simulink model "hdlcoderviterbi2"  (R2026a)
settings: Solver=VariableStepDiscrete  StopTime=8000
PreLoadFcn:
  | EsNo = 0;
libraries: commsink2 x3, commdigbbndpm3 x2, commcnvcod2 x2, commchan3 x1, commrandsrc3 x1, simulink x1
(part 1 of 2)
Description:
  | Viterbi Decoder Using the MATLAB(R) Function Block
  | This example shows how to use HDL Coder(TM) to check, generate,
  | and verify HDL for a fixed-point Viterbi decoder model built using the
  | MATLAB Function Block.
settings Model: ExtModeAutoUpdateStatusClock=off  Creator=The MathWorks, Inc.  LastModifiedBy=The MathWorks, Inc.
settings OptimizationCC: ConditionallyExecuteInputs=off  InitFltsAndDblsToZero=on  EfficientMapNaN2IntZero=off
settings DebuggingCC: AlgebraicLoopMsg=error  SignalResolutionControl=TryResolveAllWithWarning  MultiTaskDSMMsg=warning  SingleTaskRateTransMsg=error  IntegerOverflowMsg=none  ParameterPrecisionLossMsg=none  SymbolicDimsDataTypeCodeGenerationDiagnostic=none  IntegerSaturationMsg=none
settings HardwareCC: ProdHWDeviceType=ASIC/FPGA  ProdEqTarget=off
settings GRTTargetCC: CombineOutputUpdateFcns=off  GRTInterface=on

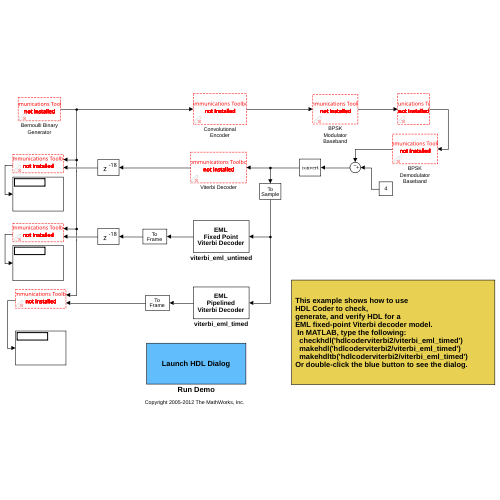
[thumbnail: Simulink's stored preview of the top-level diagram]
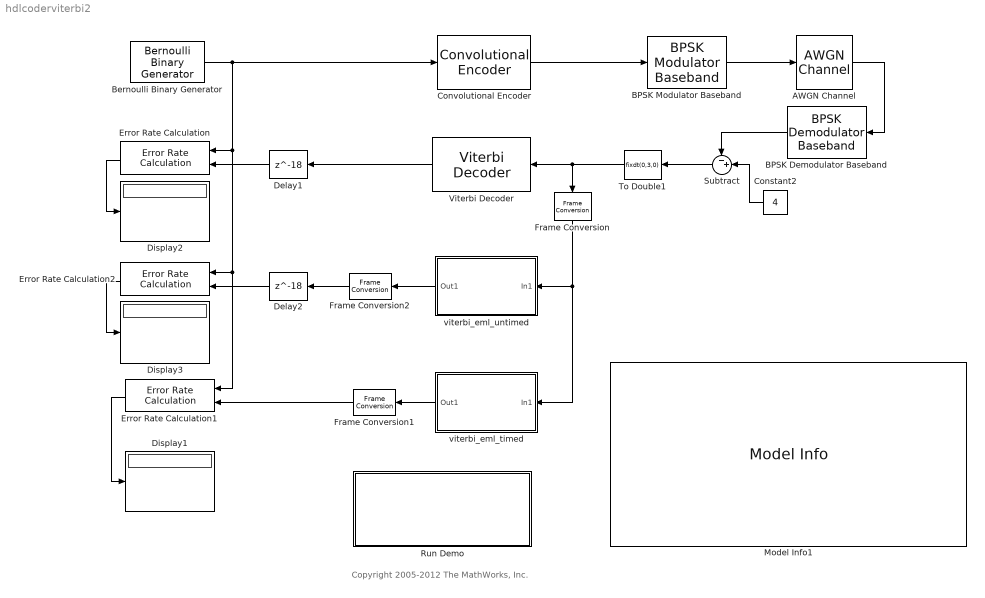
== system hdlcoderviterbi2 ==
  note: Copyright 2005-2012 The MathWorks, Inc.
  AWGN Channel : commchan3/AWGN Channel  LegacyMode=off  NoiseMethod="Signal to noise ratio  (Es/No)"  noiseMode="Signal to noise ratio  (SNR)"  EbNo=10  EsNo=EsNo  SNR=10  BitsPerSymbol=1  SignalPower=1  SamplesPerSymbol=round(0.5 / 5.000000e-01)  SymbolPeriod=0.5  VarianceSource=Parameter  Variance=1  RandomStream=mt19937ar with seed  Seed=123456  SimulateUsing=Code generation
  BPSK Demodulator Baseband : commdigbbndpm3/BPSK Demodulator Baseband  DecType=Log-likelihood ratio  VarSource=Dialog  Variance=10^(-0.1*EsNo)  Ph=0  outDtype=double  derotateFactorWordLen=16  derotateFactorDataTypeStr=Inherit: Same word length as input  derotateFactorLastDataTypeStr=Inherit: Same word length as input
  BPSK Modulator Baseband : commdigbbndpm3/BPSK Modulator Baseband  Ph=0  outDtype=double  outWordLen=16  outUDDataType=sfix(16)  outFracLenMode=Best precision  outFracLen=15  outDataTypeStr=double  outLastDataTypeStr=double
  Bernoulli Binary Generator : commrandsrc3/Bernoulli Binary Generator  ProbabilityOfZero=0.5  SeedSource=Parameter  Seed=610  SampleTime=1  SamplesPerFrame=1  OutputDataType=boolean  SimulateUsing=Interpreted execution
  Constant2 : Constant  Value=4  OutDataTypeStr=Inherit: Inherit via back propagation
  Convolutional Encoder : commcnvcod2/Convolutional Encoder  trellis=poly2trellis(7, [171 133])  opMode=Continuous  DelayedResetAction=off  hasIniStPort=off  hasFinStPort=off  usePuncVector=off  punctureVector=[1; 1; 0; 1; 0; 1]  reset=Unused parameter value
  Delay1 : Delay  DelayLength=18  InitialCondition=0  InputProcessing=Columns as channels (frame based)
  Delay2 : Delay  DelayLength=18  InitialCondition=0  InputProcessing=Columns as channels (frame based)
  Display1 : Display
  Display2 : Display
  Display3 : Display
  Error Rate Calculation : commsink2/Error Rate Calculation  N=50  st_delay=100  cp_mode=Entire frame  subframe=[]  PMode=Port  WsName=BER_Data  RsMode2=off  stop=off  numErr=500  maxBits=1e6
  Error Rate Calculation1 : commsink2/Error Rate Calculation  N=50  st_delay=100  cp_mode=Entire frame  subframe=[]  PMode=Port  WsName=BER_Data  RsMode2=off  stop=off  numErr=100  maxBits=1e7
  Error Rate Calculation2 : commsink2/Error Rate Calculation  N=50  st_delay=100  cp_mode=Entire frame  subframe=[]  PMode=Port  WsName=BER_Data  RsMode2=off  stop=off  numErr=100  maxBits=1e7
  Frame Conversion : FrameConversion  OutFrame=Sample-based
  Frame Conversion1 : FrameConversion
  Frame Conversion2 : FrameConversion
  Model Info1 : simulink/Model-Wide Utilities/Model Info  Frame=on  DisplayStringWithTags=|  HorizontalTextAlignment=Left  LeftAlignmentValue=0.02
      | This example shows how to use
      | HDL Coder to check, 
      | generate, and verify HDL for a
      | EML fixed-point Viterbi decoder model.
      |  In MATLAB, type the following:
      |   checkhdl('hdlcoderviterbi2/viterbi_eml_timed')
      |   makehdl('hdlcoderviterbi2/viterbi_eml_timed')
      |   makehdltb('hdlcoderviterbi2/viterbi_eml_timed')
      | Or double-click the blue button to see the dialog.
  Run Demo : Subsystem
      settings: OpenFcn=hdldialog(bdroot)
      mask Display: disp('Launch HDL Dialog')
  Subtract : Sum  Inputs=-+|
  To Double1 : DataTypeConversion  OutDataTypeStr=fixdt(0,3,0)
  Viterbi Decoder : commcnvcod2/Viterbi Decoder  trellis=poly2trellis(7, [171 133])  isPunctured=off  punctureVector=[1; 1; 0; 1; 0; 1]  erasures=off  dectype=Soft decision  nsdecb=3  runSigValErrCheck=off  tbdepth=32  opmode=Continuous  reset=off  delayedResetAction=off  smWordLength=16  outDataType=boolean
  viterbi_eml_timed : Subsystem
      settings: RTWMemSecFuncInitTerm=Default  RTWMemSecFuncExecute=Default  RTWMemSecDataConstants=Default  RTWMemSecDataInternal=Default  RTWMemSecDataParameters=Default
      mask Display: disp('EML\nPipelined\nViterbi Decoder');
  viterbi_eml_untimed : Subsystem
      settings: RTWMemSecFuncInitTerm=Default  RTWMemSecFuncExecute=Default  RTWMemSecDataConstants=Default  RTWMemSecDataInternal=Default  RTWMemSecDataParameters=Default
      mask Display: disp('EML\nFixed Point\nViterbi Decoder');
  wires:
  Bernoulli Binary Generator/1 -> Error Rate Calculation/1, Error Rate Calculation2/1, Error Rate Calculation1/1, Convolutional Encoder/1
  BPSK Modulator Baseband/1 -> AWGN Channel/1
  Convolutional Encoder/1 -> BPSK Modulator Baseband/1
  viterbi_eml_untimed/1(Out1) -> Frame Conversion2/1
  Viterbi Decoder/1 -> Delay1/1
  Subtract/1 -> To Double1/1
  To Double1/1 -> Viterbi Decoder/1, Frame Conversion/1
  Frame Conversion/1 -> viterbi_eml_untimed/1(In1), viterbi_eml_timed/1(In1)
  Frame Conversion2/1 -> Delay2/1
  viterbi_eml_timed/1(Out1) -> Frame Conversion1/1
  Frame Conversion1/1 -> Error Rate Calculation1/2
  Delay1/1 -> Error Rate Calculation/2
  Delay2/1 -> Error Rate Calculation2/2
  Error Rate Calculation/1 -> Display2/1
  Error Rate Calculation2/1 -> Display3/1
  Error Rate Calculation1/1 -> Display1/1
  AWGN Channel/1 -> BPSK Demodulator Baseband/1
  BPSK Demodulator Baseband/1 -> Subtract/1
  Constant2/1 -> Subtract/2

== system hdlcoderviterbi2/Run Demo ==

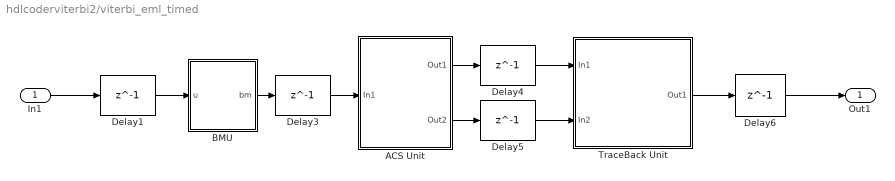
== system hdlcoderviterbi2/viterbi_eml_timed ==
  In1 : Inport
  ACS Unit : Subsystem
      settings: RTWMemSecFuncInitTerm=Default  RTWMemSecFuncExecute=Default  RTWMemSecDataConstants=Default  RTWMemSecDataInternal=Default  RTWMemSecDataParameters=Default
  BMU : MATLAB Function  TreatAsAtomicUnit=on
  Delay{1,3..6} (5 alike) : Delay  DelayLength=1  InitialCondition=0  UseCircularBuffer=on
  TraceBack Unit : Subsystem
  Out1 : Outport  VectorParamsAs1DForOutWhenUnconnected=off
  wires:
  In1/1 -> Delay1/1
  ACS Unit/1(Out1) -> Delay4/1
  ACS Unit/2(Out2) -> Delay5/1
  TraceBack Unit/1(Out1) -> Delay6/1
  BMU/1(bm) -> Delay3/1
  Delay1/1 -> BMU/1(u)
  Delay3/1 -> ACS Unit/1(In1)
  Delay4/1 -> TraceBack Unit/1(In1)
  Delay5/1 -> TraceBack Unit/2(In2)
  Delay6/1 -> Out1/1

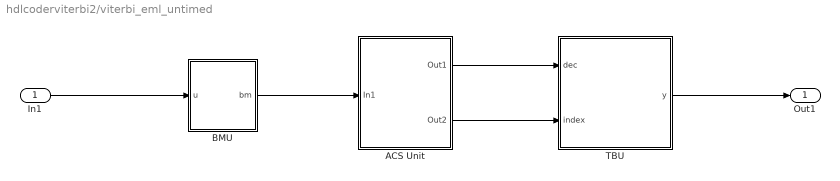
== system hdlcoderviterbi2/viterbi_eml_untimed ==
  In1 : Inport
  ACS Unit : Subsystem
      settings: RTWMemSecFuncInitTerm=Default  RTWMemSecFuncExecute=Default  RTWMemSecDataConstants=Default  RTWMemSecDataInternal=Default  RTWMemSecDataParameters=Default
  BMU : MATLAB Function  TreatAsAtomicUnit=on
  TBU : MATLAB Function  TreatAsAtomicUnit=on
  Out1 : Outport  VectorParamsAs1DForOutWhenUnconnected=off
  wires:
  In1/1 -> BMU/1(u)
  ACS Unit/1(Out1) -> TBU/1(dec)
  ACS Unit/2(Out2) -> TBU/2(index)
  TBU/1(y) -> Out1/1
  BMU/1(bm) -> ACS Unit/1(In1)

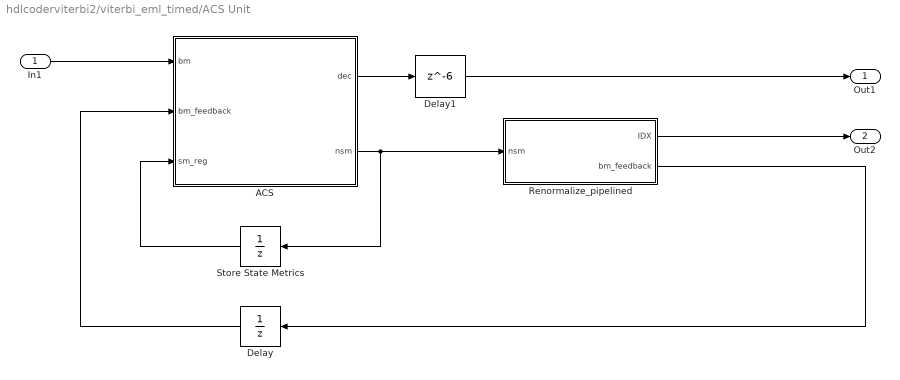
== system hdlcoderviterbi2/viterbi_eml_timed/ACS Unit ==
  In1 : Inport
  ACS : MATLAB Function  TreatAsAtomicUnit=on
  Delay : UnitDelay  SampleTime=-1
  Delay1 : Delay  DelayLength=6  InitialCondition=0
  Renormalize_pipelined : MATLAB Function  TreatAsAtomicUnit=on
  Store State Metrics : UnitDelay  SampleTime=-1
  Out1 : Outport  VectorParamsAs1DForOutWhenUnconnected=off
  Out2 : Outport  Port=2  VectorParamsAs1DForOutWhenUnconnected=off
  wires:
  Store State Metrics/1 -> ACS/3(sm_reg)
  ACS/1(dec) -> Delay1/1
  Delay/1 -> ACS/2(bm_feedback)
  In1/1 -> ACS/1(bm)
  ACS/2(nsm) -> Store State Metrics/1, Renormalize_pipelined/1(nsm)
  Renormalize_pipelined/2(bm_feedback) -> Delay/1
  Delay1/1 -> Out1/1
  Renormalize_pipelined/1(IDX) -> Out2/1

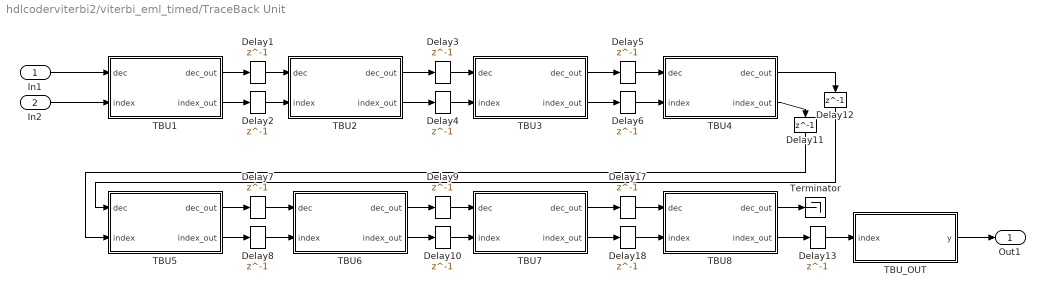
== system hdlcoderviterbi2/viterbi_eml_timed/TraceBack Unit ==
  In1 : Inport
  In2 : Inport  Port=2
  Delay{1..13,17..18} (15 alike) : Delay  DelayLength=1  InitialCondition=0  UseCircularBuffer=on
  TBU1 : MATLAB Function  TreatAsAtomicUnit=on
  TBU2 : MATLAB Function  TreatAsAtomicUnit=on
  TBU3 : MATLAB Function  TreatAsAtomicUnit=on
  TBU4 : MATLAB Function  TreatAsAtomicUnit=on
  TBU5 : MATLAB Function  TreatAsAtomicUnit=on
  TBU6 : MATLAB Function  TreatAsAtomicUnit=on
  TBU7 : MATLAB Function  TreatAsAtomicUnit=on
  TBU8 : MATLAB Function  TreatAsAtomicUnit=on
  TBU_OUT : MATLAB Function  TreatAsAtomicUnit=on
  Terminator : Terminator
  Out1 : Outport  VectorParamsAs1DForOutWhenUnconnected=off
  wires:
  In1/1 -> TBU1/1(dec)
  In2/1 -> TBU1/2(index)
  TBU4/2(index_out) -> Delay11/1
  TBU4/1(dec_out) -> Delay12/1
  TBU1/1(dec_out) -> Delay1/1
  TBU1/2(index_out) -> Delay2/1
  Delay1/1 -> TBU2/1(dec)
  Delay2/1 -> TBU2/2(index)
  Delay3/1 -> TBU3/1(dec)
  Delay4/1 -> TBU3/2(index)
  TBU2/1(dec_out) -> Delay3/1
  TBU2/2(index_out) -> Delay4/1
  TBU3/1(dec_out) -> Delay5/1
  TBU3/2(index_out) -> Delay6/1
  Delay5/1 -> TBU4/1(dec)
  Delay6/1 -> TBU4/2(index)
  TBU5/1(dec_out) -> Delay7/1
  TBU5/2(index_out) -> Delay8/1
  Delay7/1 -> TBU6/1(dec)
  Delay8/1 -> TBU6/2(index)
  Delay9/1 -> TBU7/1(dec)
  Delay10/1 -> TBU7/2(index)
  TBU6/1(dec_out) -> Delay9/1
  TBU6/2(index_out) -> Delay10/1
  TBU7/1(dec_out) -> Delay17/1
  TBU7/2(index_out) -> Delay18/1
  Delay17/1 -> TBU8/1(dec)
  Delay18/1 -> TBU8/2(index)
  Delay12/1 -> TBU5/1(dec)
  Delay11/1 -> TBU5/2(index)
  TBU8/1(dec_out) -> Terminator/1
  TBU8/2(index_out) -> Delay13/1
  Delay13/1 -> TBU_OUT/1(index)
  TBU_OUT/1(y) -> Out1/1

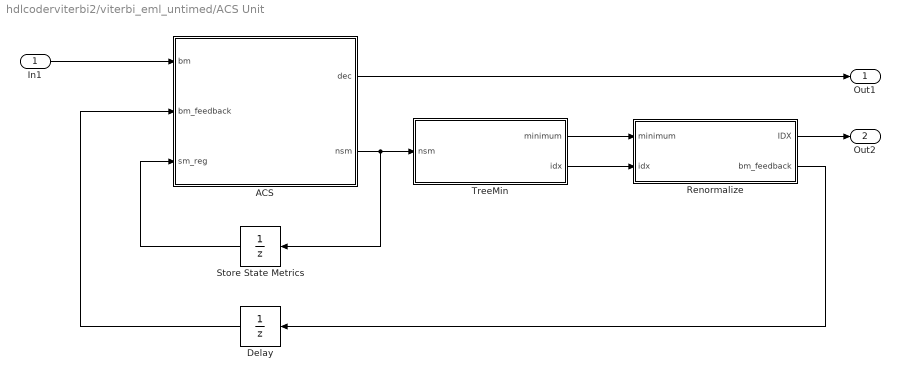
== system hdlcoderviterbi2/viterbi_eml_untimed/ACS Unit ==
  In1 : Inport
  ACS : MATLAB Function  TreatAsAtomicUnit=on
  Delay : UnitDelay  SampleTime=-1
  Renormalize : MATLAB Function  TreatAsAtomicUnit=on
  Store State Metrics : UnitDelay  SampleTime=-1
  TreeMin : MATLAB Function  TreatAsAtomicUnit=on
  Out1 : Outport  VectorParamsAs1DForOutWhenUnconnected=off
  Out2 : Outport  Port=2  VectorParamsAs1DForOutWhenUnconnected=off
  wires:
  Store State Metrics/1 -> ACS/3(sm_reg)
  ACS/1(dec) -> Out1/1
  Delay/1 -> ACS/2(bm_feedback)
  In1/1 -> ACS/1(bm)
  TreeMin/1(minimum) -> Renormalize/1(minimum)
  Renormalize/1(IDX) -> Out2/1
  ACS/2(nsm) -> TreeMin/1(nsm), Store State Metrics/1
  Renormalize/2(bm_feedback) -> Delay/1
  TreeMin/2(idx) -> Renormalize/2(idx)

== matlab function hdlcoderviterbi2/viterbi_eml_untimed/TBU ==
  settings: fimath=|
      | fimath(...
      | 'RoundMode', 'floor',...
      | 'OverflowMode', 'wrap',...
      | 'ProductMode', 'FullPrecision', 'ProductWordLength', 32,...
      | 'SumMode', 'FullPrecision', 'SumWordLength', 32,...
      | 'CastBeforeSum', true)
  data: dec input fixdt(0,1,0) size=[1 64]; index input fixdt(0,8,0) size=1; y output
function y = TBU(dec, index)

% traceback storage register
persistent tb_reg;  
if isempty(tb_reg)
    tb_reg = getfi(zeros(1,64), 0, 32, 0);
end

   
%--------------------------------------------------------------------------
% TBU (Trace Back Unit)
% Trace back unit restore the optimal path information stored in the 
% path metric register. The trace back depth of this decoder is 32 steps,
% which means every decoded symbol is based on the minimum path metric in the
% following 32 steps. 
%
% The trace back unit is implemented by a 32 stage shift register.
% Normal implementation uses 32 64-bit registers for trance back unit. 
% We use 64 32-bit registers instead because of the fixed-point bitwidth limit.
%--------------------------------------------------------------------------

% stores path metric decision inforamtion from PMU unit
tb_reg = bitconcat(bitsliceget(tb_reg, 31, 1), dec);

% trace back unit
for i=1:32
  index = tbunit(index, tb_reg, i);
end

% the 6th bit of the 32th trace back step is the decoder output
tband = bitget(index, 6);
y =  logical(tband);

end

%--------------------------------------------------------------------------
% TB Unit (Trace Back Unit)
% Given the index of the minimum metric node in the current stages,
% also given the stored decision information in the current stages,
% we can restore the index of the minimum metric node in the previous stage.
%--------------------------------------------------------------------------
function new_idx = tbunit (current_idx, tb_reg, stage)

idx = int32(current_idx) + int32(1);
tbread = bitget(tb_reg(idx), stage);

shift_idx = bitconcat(bitsliceget(current_idx, 5, 1), tbread);
new_idx = bitconcat(getfi(0, 0, 2, 0), shift_idx);

end


function myfi = getfi(input, issigned, wlen, flen)

fm = fimath(...
    'RoundMode', 'floor',...
    'OverflowMode', 'wrap',...
    'ProductMode', 'FullPrecision', 'ProductWordLength', 32,...
    'SumMode', 'FullPrecision', 'SumWordLength', 32,...
    'CastBeforeSum', true);

myfi = fi(input, issigned, wlen, flen, 'fimath', fm);

end

== matlab function hdlcoderviterbi2/viterbi_eml_timed/BMU ==
  settings: fimath=|
      | fimath(...
      | 'RoundMode', 'floor',...
      | 'OverflowMode', 'wrap',...
      | 'ProductMode', 'FullPrecision', 'ProductWordLength', 32,...
      | 'SumMode', 'FullPrecision', 'SumWordLength', 32,...
      | 'CastBeforeSum', true)
  data: u input fixdt(0,3,0) size=2; bm output
function bm = BMU(u)
%--------------------------------------------------------------------------
% Viterbi Decoder Demo
% 
% This model implements viterbi decoder in MATLAB Coder.
% The Viterbi Decoder block decodes fixed-point input symbols to produce 
% binary output symbols.
%--------------------------------------------------------------------------

% input symbol
u1 = u(1);
u2 = u(2);

%--------------------------------------------------------------------------
% BMC (Branch Metric) Unit
% This block calculates the Branch Metric (Hamming distance) of input symbols.
% The input are the quantized fixed-point symbols in the form of ufix3.

% Input Value   Interpretation
% 
% 0          Most confident zero
% 1          Second most confident zero
% 2          Third most confident zero
% 3          Least confident zero
% 4          Least confident one
% 5          Third most confident one
% 6          Second most confident one
% 7          Most confident one

%--------------------------------------------------------------------------

bm_max = getfi(7, 0, 3, 0);

bm_t1 = getfi(bm_max - u1, 0, 3, 0);
bm_t2 = getfi(bm_max - u2, 0, 3, 0);

bm = getfi(zeros(1,4), 0, 4, 0);

%----------------------------
bm(1) = u1 + u2; 

%----------------------------
bm(2) = u1 + bm_t2; 

%----------------------------
bm(3) = bm_t1 + u2;

%----------------------------
bm(4) = bm_t1 + bm_t2;

end

function myfi = getfi(input, issigned, wlen, flen)

fm = fimath(...
    'RoundMode', 'floor',...
    'OverflowMode', 'wrap',...
    'ProductMode', 'FullPrecision', 'ProductWordLength', 32,...
    'SumMode', 'FullPrecision', 'SumWordLength', 32,...
    'CastBeforeSum', true);

myfi = fi(input, issigned, wlen, flen, 'fimath', fm);

end

== matlab function hdlcoderviterbi2/viterbi_eml_timed/TraceBack Unit/TBU1 ==
  settings: fimath=|
      | fimath(...
      | 'RoundMode', 'floor',...
      | 'OverflowMode', 'wrap',...
      | 'ProductMode', 'FullPrecision', 'ProductWordLength', 32,...
      | 'SumMode', 'FullPrecision', 'SumWordLength', 32,...
      | 'CastBeforeSum', true)
  data: dec input fixdt(0,1,0) size=[1 64]; index input fixdt(0,8,0) size=1; dec_out output; index_out output
function [dec_out, index_out] = TBU(dec, index)
%--------------------------------------------------------------------------
% TBU (Trace Back Unit)
% Trace back unit restore the optimal path information stored in the 
% path metric register. The trace back depth of this decoder is 32 steps,
% which means every decoded symbol is based on the minimum path metric in the
% following 32 steps. 
%
% The trace back unit is implemented by a 32 stage shift register.
% In this pipelined model, 32 stage shift register is breaked into 8 4-stage shift registers. 
%--------------------------------------------------------------------------

% initialize 4-stage trace back storage shift register
persistent tb_reg1 tb_reg2 tb_reg3 tb_reg4
if isempty(tb_reg1)
    tb_reg1 = getfi(zeros(1, 64), 0, 1, 0);
end
if isempty(tb_reg2)
    tb_reg2 = getfi(zeros(1, 64), 0, 1, 0);
end
if isempty(tb_reg3)
    tb_reg3 = getfi(zeros(1, 64), 0, 1, 0);
end
if isempty(tb_reg4)
    tb_reg4 = getfi(zeros(1, 64), 0, 1, 0);
end

% 4-stage trace back storage shift register
% stores path metric decision inforamtion from ACS unit
dec_out = tb_reg4;
tb_reg4 = tb_reg3;
tb_reg3 = tb_reg2;
tb_reg2 = tb_reg1;
tb_reg1 = dec;

% stage one
idx = int32(index) + int32(1);
tbread = tb_reg1(idx);
shift_idx = bitconcat(bitsliceget(index, 5, 1), tbread);
index = bitconcat(getfi(0, 0, 2, 0), shift_idx);

% stage two
idx = int32(index) + int32(1);
tbread = tb_reg2(idx);
shift_idx = bitconcat(bitsliceget(index, 5, 1), tbread);
index = bitconcat(getfi(0, 0, 2, 0), shift_idx);

% stage three
idx = int32(index) + int32(1);
tbread = tb_reg3(idx);
shift_idx = bitconcat(bitsliceget(index, 5, 1), tbread);
index = bitconcat(getfi(0, 0, 2, 0), shift_idx);

% stage four
idx = int32(index) + int32(1);
tbread = tb_reg4(idx);
shift_idx = bitconcat(bitsliceget(index, 5, 1), tbread);
index_out = bitconcat(getfi(0, 0, 2, 0), shift_idx);

end

function myfi = getfi(input, issigned, wlen, flen)

fm = fimath(...
    'RoundMode', 'floor',...
    'OverflowMode', 'wrap',...
    'ProductMode', 'FullPrecision', 'ProductWordLength', 32,...
    'SumMode', 'FullPrecision', 'SumWordLength', 32,...
    'CastBeforeSum', true);

myfi = fi(input, issigned, wlen, flen, 'fimath', fm);

end

== matlab function hdlcoderviterbi2/viterbi_eml_timed/TraceBack Unit/TBU6 ==
  settings: fimath=|
      | fimath(...
      | 'RoundMode', 'floor',...
      | 'OverflowMode', 'wrap',...
      | 'ProductMode', 'FullPrecision', 'ProductWordLength', 32,...
      | 'SumMode', 'FullPrecision', 'SumWordLength', 32,...
      | 'CastBeforeSum', true)
  data: dec input fixdt(0,1,0) size=[1 64]; index input fixdt(0,8,0) size=1; dec_out output; index_out output
function [dec_out, index_out] = TBU(dec, index)
%--------------------------------------------------------------------------
% TBU (Trace Back Unit)
% Trace back unit restore the optimal path information stored in the 
% path metric register. The trace back depth of this decoder is 32 steps,
% which means every decoded symbol is based on the minimum path metric in the
% following 32 steps. 
%
% The trace back unit is implemented by a 32 stage shift register.
% In this pipelined model, 32 stage shift register is breaked into 8 4-stage shift registers. 
%--------------------------------------------------------------------------

% initialize 4-stage trace back storage shift register
persistent tb_reg1 tb_reg2 tb_reg3 tb_reg4
if isempty(tb_reg1)
    tb_reg1 = getfi(zeros(1, 64), 0, 1, 0);
end
if isempty(tb_reg2)
    tb_reg2 = getfi(zeros(1, 64), 0, 1, 0);
end
if isempty(tb_reg3)
    tb_reg3 = getfi(zeros(1, 64), 0, 1, 0);
end
if isempty(tb_reg4)
    tb_reg4 = getfi(zeros(1, 64), 0, 1, 0);
end

% 4-stage trace back storage shift register
% stores path metric decision inforamtion from ACS unit
dec_out = tb_reg4;
tb_reg4 = tb_reg3;
tb_reg3 = tb_reg2;
tb_reg2 = tb_reg1;
tb_reg1 = dec;

% stage one
idx = int32(index) + int32(1);
tbread = tb_reg1(idx);
shift_idx = bitconcat(bitsliceget(index, 5, 1), tbread);
index = bitconcat(getfi(0, 0, 2, 0), shift_idx);

% stage two
idx = int32(index) + int32(1);
tbread = tb_reg2(idx);
shift_idx = bitconcat(bitsliceget(index, 5, 1), tbread);
index = bitconcat(getfi(0, 0, 2, 0), shift_idx);

% stage three
idx = int32(index) + int32(1);
tbread = tb_reg3(idx);
shift_idx = bitconcat(bitsliceget(index, 5, 1), tbread);
index = bitconcat(getfi(0, 0, 2, 0), shift_idx);

% stage four
idx = int32(index) + int32(1);
tbread = tb_reg4(idx);
shift_idx = bitconcat(bitsliceget(index, 5, 1), tbread);
index_out = bitconcat(getfi(0, 0, 2, 0), shift_idx);

end

function myfi = getfi(input, issigned, wlen, flen)

fm = fimath(...
    'RoundMode', 'floor',...
    'OverflowMode', 'wrap',...
    'ProductMode', 'FullPrecision', 'ProductWordLength', 32,...
    'SumMode', 'FullPrecision', 'SumWordLength', 32,...
    'CastBeforeSum', true);

myfi = fi(input, issigned, wlen, flen, 'fimath', fm);

end

== matlab function hdlcoderviterbi2/viterbi_eml_timed/TraceBack Unit/TBU7 ==
  settings: fimath=|
      | fimath(...
      | 'RoundMode', 'floor',...
      | 'OverflowMode', 'wrap',...
      | 'ProductMode', 'FullPrecision', 'ProductWordLength', 32,...
      | 'SumMode', 'FullPrecision', 'SumWordLength', 32,...
      | 'CastBeforeSum', true)
  data: dec input fixdt(0,1,0) size=[1 64]; index input fixdt(0,8,0) size=1; dec_out output; index_out output
function [dec_out, index_out] = TBU(dec, index)
%--------------------------------------------------------------------------
% TBU (Trace Back Unit)
% Trace back unit restore the optimal path information stored in the 
% path metric register. The trace back depth of this decoder is 32 steps,
% which means every decoded symbol is based on the minimum path metric in the
% following 32 steps. 
%
% The trace back unit is implemented by a 32 stage shift register.
% In this pipelined model, 32 stage shift register is breaked into 8 4-stage shift registers. 
%--------------------------------------------------------------------------

% initialize 4-stage trace back storage shift register
persistent tb_reg1 tb_reg2 tb_reg3 tb_reg4
if isempty(tb_reg1)
    tb_reg1 = getfi(zeros(1, 64), 0, 1, 0);
end
if isempty(tb_reg2)
    tb_reg2 = getfi(zeros(1, 64), 0, 1, 0);
end
if isempty(tb_reg3)
    tb_reg3 = getfi(zeros(1, 64), 0, 1, 0);
end
if isempty(tb_reg4)
    tb_reg4 = getfi(zeros(1, 64), 0, 1, 0);
end

% 4-stage trace back storage shift register
% stores path metric decision inforamtion from ACS unit
dec_out = tb_reg4;
tb_reg4 = tb_reg3;
tb_reg3 = tb_reg2;
tb_reg2 = tb_reg1;
tb_reg1 = dec;

% stage one
idx = int32(index) + int32(1);
tbread = tb_reg1(idx);
shift_idx = bitconcat(bitsliceget(index, 5, 1), tbread);
index = bitconcat(getfi(0, 0, 2, 0), shift_idx);

% stage two
idx = int32(index) + int32(1);
tbread = tb_reg2(idx);
shift_idx = bitconcat(bitsliceget(index, 5, 1), tbread);
index = bitconcat(getfi(0, 0, 2, 0), shift_idx);

% stage three
idx = int32(index) + int32(1);
tbread = tb_reg3(idx);
shift_idx = bitconcat(bitsliceget(index, 5, 1), tbread);
index = bitconcat(getfi(0, 0, 2, 0), shift_idx);

% stage four
idx = int32(index) + int32(1);
tbread = tb_reg4(idx);
shift_idx = bitconcat(bitsliceget(index, 5, 1), tbread);
index_out = bitconcat(getfi(0, 0, 2, 0), shift_idx);

end

function myfi = getfi(input, issigned, wlen, flen)

fm = fimath(...
    'RoundMode', 'floor',...
    'OverflowMode', 'wrap',...
    'ProductMode', 'FullPrecision', 'ProductWordLength', 32,...
    'SumMode', 'FullPrecision', 'SumWordLength', 32,...
    'CastBeforeSum', true);

myfi = fi(input, issigned, wlen, flen, 'fimath', fm);

end

== matlab function hdlcoderviterbi2/viterbi_eml_timed/TraceBack Unit/TBU8 ==
  settings: fimath=|
      | fimath(...
      | 'RoundMode', 'floor',...
      | 'OverflowMode', 'wrap',...
      | 'ProductMode', 'FullPrecision', 'ProductWordLength', 32,...
      | 'SumMode', 'FullPrecision', 'SumWordLength', 32,...
      | 'CastBeforeSum', true)
  data: dec input fixdt(0,1,0) size=[1 64]; index input fixdt(0,8,0) size=1; dec_out output; index_out output
function [dec_out, index_out] = TBU(dec, index)
%--------------------------------------------------------------------------
% TBU (Trace Back Unit)
% Trace back unit restore the optimal path information stored in the 
% path metric register. The trace back depth of this decoder is 32 steps,
% which means every decoded symbol is based on the minimum path metric in the
% following 32 steps. 
%
% The trace back unit is implemented by a 32 stage shift register.
% In this pipelined model, 32 stage shift register is breaked into 8 4-stage shift registers. 
%--------------------------------------------------------------------------

% initialize 4-stage trace back storage shift register
persistent tb_reg1 tb_reg2 tb_reg3 tb_reg4
if isempty(tb_reg1)
    tb_reg1 = getfi(zeros(1, 64), 0, 1, 0);
end
if isempty(tb_reg2)
    tb_reg2 = getfi(zeros(1, 64), 0, 1, 0);
end
if isempty(tb_reg3)
    tb_reg3 = getfi(zeros(1, 64), 0, 1, 0);
end
if isempty(tb_reg4)
    tb_reg4 = getfi(zeros(1, 64), 0, 1, 0);
end

% 4-stage trace back storage shift register
% stores path metric decision inforamtion from ACS unit
dec_out = tb_reg4;
tb_reg4 = tb_reg3;
tb_reg3 = tb_reg2;
tb_reg2 = tb_reg1;
tb_reg1 = dec;

% stage one
idx = int32(index) + int32(1);
tbread = tb_reg1(idx);
shift_idx = bitconcat(bitsliceget(index, 5, 1), tbread);
index = bitconcat(getfi(0, 0, 2, 0), shift_idx);

% stage two
idx = int32(index) + int32(1);
tbread = tb_reg2(idx);
shift_idx = bitconcat(bitsliceget(index, 5, 1), tbread);
index = bitconcat(getfi(0, 0, 2, 0), shift_idx);

% stage three
idx = int32(index) + int32(1);
tbread = tb_reg3(idx);
shift_idx = bitconcat(bitsliceget(index, 5, 1), tbread);
index = bitconcat(getfi(0, 0, 2, 0), shift_idx);

% stage four
idx = int32(index) + int32(1);
tbread = tb_reg4(idx);
shift_idx = bitconcat(bitsliceget(index, 5, 1), tbread);
index_out = bitconcat(getfi(0, 0, 2, 0), shift_idx);

end

function myfi = getfi(input, issigned, wlen, flen)

fm = fimath(...
    'RoundMode', 'floor',...
    'OverflowMode', 'wrap',...
    'ProductMode', 'FullPrecision', 'ProductWordLength', 32,...
    'SumMode', 'FullPrecision', 'SumWordLength', 32,...
    'CastBeforeSum', true);

myfi = fi(input, issigned, wlen, flen, 'fimath', fm);

end

== matlab function hdlcoderviterbi2/viterbi_eml_timed/TraceBack Unit/TBU_OUT ==
  settings: fimath=|
      | fimath(...
      | 'RoundMode', 'floor',...
      | 'OverflowMode', 'wrap',...
      | 'ProductMode', 'FullPrecision', 'ProductWordLength', 32,...
      | 'SumMode', 'FullPrecision', 'SumWordLength', 32,...
      | 'CastBeforeSum', true)
  data: index input fixdt(0,8,0) size=1; y output
function y = TBU_OUT(index)

% the 6th bit of the 32th trace back step is the decoder output
tband = bitget(index, 6);
y =  logical(tband);

end

== matlab function hdlcoderviterbi2/viterbi_eml_untimed/ACS Unit/TreeMin ==
  settings: fimath=|
      | fimath(...
      |     'RoundMode', 'floor',...
      |     'OverflowMode', 'wrap',...
      |     'ProductMode', 'FullPrecision', 'ProductWordLength', 32,...
      |     'SumMode', 'FullPrecision', 'SumWordLength', 32,...
      |     'CastBeforeSum', true);
  data: minimum output; idx output uint8; nsm input fixdt(0,7,0) size=[1 64]
function [minimum, idx]  = TreeMin(nsm)
%--------------------------------------------------------------------------
% Tree implementation min function for vector input of length 64
%--------------------------------------------------------------------------

% reverse the order of input vector
nsm_reverse = nsm(64:-1:1);

% use tree_min 
[minimum, idx] = tree_min(nsm_reverse);

end

%---------------------------
function [minval, finalidx] = tree_min(invec)

% first level of comparison
inidx = int32(1:64);
[lvlonemin, lvloneidx] = vector_min(invec, inidx);

% second level of comparison
[lvltwomin, lvltwoidx] = vector_min(lvlonemin, lvloneidx);

% third level of comparison
[lvlthreemin, lvlthreeidx] = vector_min(lvltwomin, lvltwoidx);

% fourth level of comparison
[lvlfourmin, lvlfouridx] = vector_min(lvlthreemin, lvlthreeidx);

% fifth level of comparison
[lvlfivemin, lvlfiveidx] = vector_min(lvlfourmin, lvlfouridx);

% final comparison
[minval, idx] = vector_min(lvlfivemin, lvlfiveidx);

finalidx = uint8(idx);

end

% Minimum subfuction for tree implementation
function [minvec, idxvec] = vector_min(invec, inidx)
    
lengthminvec = bitshift(uint8(length(invec)), -1);
minvec = getfi(zeros(1, lengthminvec), 0, 7, 0);
idxvec = int32(zeros(1, lengthminvec));

for i=int32(1:lengthminvec)
    % get two consecutive values
    idx2 = int32(i)+int32(i); %i*2
    idx1 = int32(idx2) - int32(1); %i*2-1
    % get elements
    val1 = invec(idx1);
    val2 = invec(idx2);
    % compare them and select minimum
    if val1 <= val2
        minvec(i) = val1;
        idxvec(i) = inidx(idx1);
    else
        minvec(i) = val2;
        idxvec(i) = inidx(idx2);
    end
end

end


function myfi = getfi(input, issigned, wlen, flen)

fm = fimath(...
    'RoundMode', 'floor',...
    'OverflowMode', 'wrap',...
    'ProductMode', 'FullPrecision', 'ProductWordLength', 32,...
    'SumMode', 'FullPrecision', 'SumWordLength', 32,...
    'CastBeforeSum', true);

myfi = fi(input, issigned, wlen, flen, 'fimath', fm);

end

== matlab function hdlcoderviterbi2/viterbi_eml_untimed/ACS Unit/Renormalize ==
  settings: fimath=|
      | fimath(...
      |     'RoundMode', 'floor',...
      |     'OverflowMode', 'saturate',...
      |     'ProductMode', 'FullPrecision', 'ProductWordLength', 32,...
      |     'SumMode', 'FullPrecision', 'SumWordLength', 32,...
      |     'CastBeforeSum', true);
  data: minimum input fixdt(0,7,0); idx input uint8; IDX output; bm_feedback output size=1
function [IDX, bm_feedback]  = Renormalize(minimum, idx)

%--------------------------------------------------------------------------
% Renormalize Block
% Finds the state with minimum path metric and outputs its index
% Then renormalizes all the path metrics by subsracting the minimum metric
%--------------------------------------------------------------------------

if minimum < 32
    bm_feedback = getfi(0, 0, 7, 0);
else
    bm_feedback = getfi(112, 0, 7, 0);
end
    
index = getfi((idx-1), 0, 8, 0);
index_max = getfi(63, 0, 8, 0);
IDX = getfi(index_max - index, 0, 8, 0);
    
end


function myfi = getfi(input, issigned, wlen, flen)

fm = fimath(...
    'RoundMode', 'floor',...
    'OverflowMode', 'wrap',...
    'ProductMode', 'FullPrecision', 'ProductWordLength', 32,...
    'SumMode', 'FullPrecision', 'SumWordLength', 32,...
    'CastBeforeSum', true);

myfi = fi(input, issigned, wlen, flen, 'fimath', fm);

end

== matlab function hdlcoderviterbi2/viterbi_eml_untimed/BMU ==
  settings: fimath=|
      | fimath(...
      | 'RoundMode', 'floor',...
      | 'OverflowMode', 'wrap',...
      | 'ProductMode', 'FullPrecision', 'ProductWordLength', 32,...
      | 'SumMode', 'FullPrecision', 'SumWordLength', 32,...
      | 'CastBeforeSum', true)
  data: u input fixdt(0,3,0) size=2; bm output
function bm = BMU(u)
%--------------------------------------------------------------------------
% Viterbi Decoder Demo
% 
% This model implements viterbi decoder in MATLAB Coder.
% The Viterbi Decoder block decodes fixed-point input symbols to produce 
% binary output symbols.
%--------------------------------------------------------------------------

% input symbol
u1 = u(1);
u2 = u(2);

%--------------------------------------------------------------------------
% BMC (Branch Metric) Unit
% This block calculates the Branch Metric (Hamming distance) of input symbols.
% The input are the quantized fixed-point symbols in the form of ufix3.

% Input Value   Interpretation
% 
% 0          Most confident zero
% 1          Second most confident zero
% 2          Third most confident zero
% 3          Least confident zero
% 4          Least confident one
% 5          Third most confident one
% 6          Second most confident one
% 7          Most confident one

%--------------------------------------------------------------------------

bm_max = getfi(7, 0, 3, 0);

bm_t1 = getfi(bm_max - u1, 0, 3, 0);
bm_t2 = getfi(bm_max - u2, 0, 3, 0);

bm = getfi(zeros(1,4), 0, 4, 0);

%----------------------------
bm(1) = u1 + u2; 

%----------------------------
bm(2) = u1 + bm_t2; 

%----------------------------
bm(3) = bm_t1 + u2;

%----------------------------
bm(4) = bm_t1 + bm_t2;

end

function myfi = getfi(input, issigned, wlen, flen)

fm = fimath(...
    'RoundMode', 'floor',...
    'OverflowMode', 'wrap',...
    'ProductMode', 'FullPrecision', 'ProductWordLength', 32,...
    'SumMode', 'FullPrecision', 'SumWordLength', 32,...
    'CastBeforeSum', true);

myfi = fi(input, issigned, wlen, flen, 'fimath', fm);

end

== matlab function hdlcoderviterbi2/viterbi_eml_untimed/ACS Unit/ACS ==
  settings: fimath=|
      | fimath(...
      |     'RoundMode', 'floor',...
      |     'OverflowMode', 'wrap',...
      |     'ProductMode', 'FullPrecision', 'ProductWordLength', 32,...
      |     'SumMode', 'FullPrecision', 'SumWordLength', 32,...
      |     'CastBeforeSum', true);
  data: dec output; nsm output; bm input fixdt(0,4,0) size=[1 4]; bm_feedback input fixdt(0,7,0); sm_reg input fixdt(0,7,0) size=[1 64]
function [dec, nsm]  = ACSU(bm, bm_feedback, sm_reg)
%--------------------------------------------------------------------------
%  ACS (Add-Compare-Select) block
%--------------------------------------------------------------------------

bm_conv = bm + bm_feedback;

bm_adjust = getfi(bm_conv, 0, 7, 0);

[nsm, dec] = acsunitbutterfly(bm_adjust, sm_reg);
   
end

%--------------------------------------------------------------------------
% ACS Unit Group(Add-Compare-Select)
% For each state in the trellis diagram, for each node in this state:
% 1. Add the branch metric to the paths merged to this node. 
% 2. Compare all the paths merged to this road
% 3. Select the path with the minimum path metric
%--------------------------------------------------------------------------
function [nsm, dec] = acsunitbutterfly(bm, sm)

nsm = getfi(zeros(1,64),0, 7, 0);
dec = getfi(zeros(1,64),0, 1, 0);

%----------------------------------------------------
% 000000   -> 00 -> 000000   000001   -> 11 -> 000000   
%----------------------------------------------------
[nsm(1), dec(1)] = acsunit(bm(1),bm(4),sm(1),sm(2));
%----------------------------------------------------
% 000000   -> 11 -> 100000   000001   -> 00 -> 100000   
%----------------------------------------------------
[nsm(33), dec(33)] = acsunit(bm(4),bm(1),sm(1),sm(2));
%----------------------------------------------------
% 000010   -> 01 -> 000001   000011   -> 10 -> 000001   
%----------------------------------------------------
[nsm(2), dec(2)] = acsunit(bm(2),bm(3),sm(3),sm(4));
%----------------------------------------------------
% 000010   -> 10 -> 100001   000011   -> 01 -> 100001   
%----------------------------------------------------
[nsm(34), dec(34)] = acsunit(bm(3),bm(2),sm(3),sm(4));
%----------------------------------------------------
% 000100   -> 00 -> 000010   000101   -> 11 -> 000010   
%----------------------------------------------------
[nsm(3), dec(3)] = acsunit(bm(1),bm(4),sm(5),sm(6));
%----------------------------------------------------
% 000100   -> 11 -> 100010   000101   -> 00 -> 100010   
%----------------------------------------------------
[nsm(35), dec(35)] = acsunit(bm(4),bm(1),sm(5),sm(6));
%----------------------------------------------------
% 000110   -> 01 -> 000011   000111   -> 10 -> 000011   
%----------------------------------------------------
[nsm(4), dec(4)] = acsunit(bm(2),bm(3),sm(7),sm(8));
%----------------------------------------------------
% 000110   -> 10 -> 100011   000111   -> 01 -> 100011   
%----------------------------------------------------
[nsm(36), dec(36)] = acsunit(bm(3),bm(2),sm(7),sm(8));
%----------------------------------------------------
% 001000   -> 11 -> 000100   001001   -> 00 -> 000100   
%----------------------------------------------------
[nsm(5), dec(5)] = acsunit(bm(4),bm(1),sm(9),sm(10));
%----------------------------------------------------
% 001000   -> 00 -> 100100   001001   -> 11 -> 100100   
%----------------------------------------------------
[nsm(37), dec(37)] = acsunit(bm(1),bm(4),sm(9),sm(10));
%----------------------------------------------------
% 001010   -> 10 -> 000101   001011   -> 01 -> 000101   
%----------------------------------------------------
[nsm(6), dec(6)] = acsunit(bm(3),bm(2),sm(11),sm(12));
%----------------------------------------------------
% 001010   -> 01 -> 100101   001011   -> 10 -> 100101   
%----------------------------------------------------
[nsm(38), dec(38)] = acsunit(bm(2),bm(3),sm(11),sm(12));
%----------------------------------------------------
% 001100   -> 11 -> 000110   001101   -> 00 -> 000110   
%----------------------------------------------------
[nsm(7), dec(7)] = acsunit(bm(4),bm(1),sm(13),sm(14));
%----------------------------------------------------
% 001100   -> 00 -> 100110   001101   -> 11 -> 100110   
%----------------------------------------------------
[nsm(39), dec(39)] = acsunit(bm(1),bm(4),sm(13),sm(14));
%----------------------------------------------------
% 001110   -> 10 -> 000111   001111   -> 01 -> 000111   
%----------------------------------------------------
[nsm(8), dec(8)] = acsunit(bm(3),bm(2),sm(15),sm(16));
%----------------------------------------------------
% 001110   -> 01 -> 100111   001111   -> 10 -> 100111   
%----------------------------------------------------
[nsm(40), dec(40)] = acsunit(bm(2),bm(3),sm(15),sm(16));
%----------------------------------------------------
% 010000   -> 11 -> 001000   010001   -> 00 -> 001000   
%----------------------------------------------------
[nsm(9), dec(9)] = acsunit(bm(4),bm(1),sm(17),sm(18));
%----------------------------------------------------
% 010000   -> 00 -> 101000   010001   -> 11 -> 101000   
%----------------------------------------------------
[nsm(41), dec(41)] = acsunit(bm(1),bm(4),sm(17),sm(18));
%----------------------------------------------------
% 010010   -> 10 -> 001001   010011   -> 01 -> 001001   
%----------------------------------------------------
[nsm(10), dec(10)] = acsunit(bm(3),bm(2),sm(19),sm(20));
%----------------------------------------------------
% 010010   -> 01 -> 101001   010011   -> 10 -> 101001   
%----------------------------------------------------
[nsm(42), dec(42)] = acsunit(bm(2),bm(3),sm(19),sm(20));
%----------------------------------------------------
% 010100   -> 11 -> 001010   010101   -> 00 -> 001010   
%----------------------------------------------------
[nsm(11), dec(11)] = acsunit(bm(4),bm(1),sm(21),sm(22));
%----------------------------------------------------
% 010100   -> 00 -> 101010   010101   -> 11 -> 101010   
%----------------------------------------------------
[nsm(43), dec(43)] = acsunit(bm(1),bm(4),sm(21),sm(22));
%----------------------------------------------------
% 010110   -> 10 -> 001011   010111   -> 01 -> 001011   
%----------------------------------------------------
[nsm(12), dec(12)] = acsunit(bm(3),bm(2),sm(23),sm(24));
%----------------------------------------------------
% 010110   -> 01 -> 101011   010111   -> 10 -> 101011   
%----------------------------------------------------
[nsm(44), dec(44)] = acsunit(bm(2),bm(3),sm(23),sm(24));
%----------------------------------------------------
% 011000   -> 00 -> 001100   011001   -> 11 -> 001100   
%----------------------------------------------------
[nsm(13), dec(13)] = acsunit(bm(1),bm(4),sm(25),sm(26));
%----------------------------------------------------
% 011000   -> 11 -> 101100   011001   -> 00 -> 101100   
%----------------------------------------------------
[nsm(45), dec(45)] = acsunit(bm(4),bm(1),sm(25),sm(26));
%----------------------------------------------------
% 011010   -> 01 -> 001101   011011   -> 10 -> 001101   
%----------------------------------------------------
[nsm(14), dec(14)] = acsunit(bm(2),bm(3),sm(27),sm(28));
%----------------------------------------------------
% 011010   -> 10 -> 101101   011011   -> 01 -> 101101   
%----------------------------------------------------
[nsm(46), dec(46)] = acsunit(bm(3),bm(2),sm(27),sm(28));
%----------------------------------------------------
% 011100   -> 00 -> 001110   011101   -> 11 -> 001110   
%----------------------------------------------------
[nsm(15), dec(15)] = acsunit(bm(1),bm(4),sm(29),sm(30));
%----------------------------------------------------
% 011100   -> 11 -> 101110   011101   -> 00 -> 101110   
%----------------------------------------------------
[nsm(47), dec(47)] = acsunit(bm(4),bm(1),sm(29),sm(30));
%----------------------------------------------------
% 011110   -> 01 -> 001111   011111   -> 10 -> 001111   
%----------------------------------------------------
[nsm(16), dec(16)] = acsunit(bm(2),bm(3),sm(31),sm(32));
%----------------------------------------------------
% 011110   -> 10 -> 101111   011111   -> 01 -> 101111   
%----------------------------------------------------
[nsm(48), dec(48)] = acsunit(bm(3),bm(2),sm(31),sm(32));
%----------------------------------------------------
% 100000   -> 10 -> 010000   100001   -> 01 -> 010000   
%----------------------------------------------------
[nsm(17), dec(17)] = acsunit(bm(3),bm(2),sm(33),sm(34));
%----------------------------------------------------
% 100000   -> 01 -> 110000   100001   -> 10 -> 110000   
%----------------------------------------------------
[nsm(49), dec(49)] = acsunit(bm(2),bm(3),sm(33),sm(34));
%----------------------------------------------------
% 100010   -> 11 -> 010001   100011   -> 00 -> 010001   
%----------------------------------------------------
[nsm(18), dec(18)] = acsunit(bm(4),bm(1),sm(35),sm(36));
%----------------------------------------------------
% 100010   -> 00 -> 110001   100011   -> 11 -> 110001   
%----------------------------------------------------
[nsm(50), dec(50)] = acsunit(bm(1),bm(4),sm(35),sm(36));
%----------------------------------------------------
% 100100   -> 10 -> 010010   100101   -> 01 -> 010010   
%----------------------------------------------------
[nsm(19), dec(19)] = acsunit(bm(3),bm(2),sm(37),sm(38));
%----------------------------------------------------
% 100100   -> 01 -> 110010   100101   -> 10 -> 110010   
%----------------------------------------------------
[nsm(51), dec(51)] = acsunit(bm(2),bm(3),sm(37),sm(38));
%----------------------------------------------------
% 100110   -> 11 -> 010011   100111   -> 00 -> 010011   
%----------------------------------------------------
[nsm(20), dec(20)] = acsunit(bm(4),bm(1),sm(39),sm(40));
%----------------------------------------------------
% 100110   -> 00 -> 110011   100111   -> 11 -> 110011   
%----------------------------------------------------
[nsm(52), dec(52)] = acsunit(bm(1),bm(4),sm(39),sm(40));
%----------------------------------------------------
% 101000   -> 01 -> 010100   101001   -> 10 -> 010100   
%----------------------------------------------------
[nsm(21), dec(21)] = acsunit(bm(2),bm(3),sm(41),sm(42));
%----------------------------------------------------
% 101000   -> 10 -> 110100   101001   -> 01 -> 110100   
%----------------------------------------------------
[nsm(53), dec(53)] = acsunit(bm(3),bm(2),sm(41),sm(42));
%----------------------------------------------------
% 101010   -> 00 -> 010101   101011   -> 11 -> 010101   
%----------------------------------------------------
[nsm(22), dec(22)] = acsunit(bm(1),bm(4),sm(43),sm(44));
%----------------------------------------------------
% 101010   -> 11 -> 110101   101011   -> 00 -> 110101   
%----------------------------------------------------
[nsm(54), dec(54)] = acsunit(bm(4),bm(1),sm(43),sm(44));
%----------------------------------------------------
% 101100   -> 01 -> 010110   101101   -> 10 -> 010110   
%----------------------------------------------------
[nsm(23), dec(23)] = acsunit(bm(2),bm(3),sm(45),sm(46));
%----------------------------------------------------
% 101100   -> 10 -> 110110   101101   -> 01 -> 110110   
%----------------------------------------------------
[nsm(55), dec(55)] = acsunit(bm(3),bm(2),sm(45),sm(46));
%----------------------------------------------------
% 101110   -> 00 -> 010111   101111   -> 11 -> 010111   
%----------------------------------------------------
[nsm(24), dec(24)] = acsunit(bm(1),bm(4),sm(47),sm(48));
%----------------------------------------------------
% 101110   -> 11 -> 110111   101111   -> 00 -> 110111   
%----------------------------------------------------
[nsm(56), dec(56)] = acsunit(bm(4),bm(1),sm(47),sm(48));
%----------------------------------------------------
% 110000   -> 01 -> 011000   110001   -> 10 -> 011000   
%----------------------------------------------------
[nsm(25), dec(25)] = acsunit(bm(2),bm(3),sm(49),sm(50));
%----------------------------------------------------
% 110000   -> 10 -> 111000   110001   -> 01 -> 111000   
%----------------------------------------------------
[nsm(57), dec(57)] = acsunit(bm(3),bm(2),sm(49),sm(50));
%----------------------------------------------------
% 110010   -> 00 -> 011001   110011   -> 11 -> 011001   
%----------------------------------------------------
[nsm(26), dec(26)] = acsunit(bm(1),bm(4),sm(51),sm(52));
%----------------------------------------------------
% 110010   -> 11 -> 111001   110011   -> 00 -> 111001   
%----------------------------------------------------
[nsm(58), dec(58)] = acsunit(bm(4),bm(1),sm(51),sm(52));
%----------------------------------------------------
% 110100   -> 01 -> 011010   110101   -> 10 -> 011010   
%----------------------------------------------------
[nsm(27), dec(27)] = acsunit(bm(2),bm(3),sm(53),sm(54));
%----------------------------------------------------
% 110100   -> 10 -> 111010   110101   -> 01 -> 111010   
%----------------------------------------------------
[nsm(59), dec(59)] = acsunit(bm(3),bm(2),sm(53),sm(54));
%----------------------------------------------------
% 110110   -> 00 -> 011011   110111   -> 11 -> 011011   
%----------------------------------------------------
[nsm(28), dec(28)] = acsunit(bm(1),bm(4),sm(55),sm(56));
%----------------------------------------------------
% 110110   -> 11 -> 111011   110111   -> 00 -> 111011   
%----------------------------------------------------
[nsm(60), dec(60)] = acsunit(bm(4),bm(1),sm(55),sm(56));
%----------------------------------------------------
% 111000   -> 10 -> 011100   111001   -> 01 -> 011100   
%----------------------------------------------------
[nsm(29), dec(29)] = acsunit(bm(3),bm(2),sm(57),sm(58));
%----------------------------------------------------
% 111000   -> 01 -> 111100   111001   -> 10 -> 111100   
%----------------------------------------------------
[nsm(61), dec(61)] = acsunit(bm(2),bm(3),sm(57),sm(58));
%----------------------------------------------------
% 111010   -> 11 -> 011101   111011   -> 00 -> 011101   
%----------------------------------------------------
[nsm(30), dec(30)] = acsunit(bm(4),bm(1),sm(59),sm(60));
%----------------------------------------------------
% 111010   -> 00 -> 111101   111011   -> 11 -> 111101   
%----------------------------------------------------
[nsm(62), dec(62)] = acsunit(bm(1),bm(4),sm(59),sm(60));
%----------------------------------------------------
% 111100   -> 10 -> 011110   111101   -> 01 -> 011110   
%----------------------------------------------------
[nsm(31), dec(31)] = acsunit(bm(3),bm(2),sm(61),sm(62));
%----------------------------------------------------
% 111100   -> 01 -> 111110   111101   -> 10 -> 111110   
%----------------------------------------------------
[nsm(63), dec(63)] = acsunit(bm(2),bm(3),sm(61),sm(62));
%----------------------------------------------------
% 111110   -> 11 -> 011111   111111   -> 00 -> 011111   
%----------------------------------------------------
[nsm(32), dec(32)] = acsunit(bm(4),bm(1),sm(63),sm(64));
%----------------------------------------------------
% 111110   -> 00 -> 111111   111111   -> 11 -> 111111   
%----------------------------------------------------
[nsm(64), dec(64)] = acsunit(bm(1),bm(4),sm(63),sm(64));

end    
    
% ACS unit
function [select_metric, decision] = acsunit(branch_metric0, branch_metric1, stored_metric0, stored_metric1)

    % update branch0 metric
    a = getfi(branch_metric0 + stored_metric0, 0, 7, 0);

    % update branch1 metric
    b = getfi(branch_metric1 + stored_metric1, 0, 7, 0);
    
    % choose the metric
    if (a <= b)
        select_metric = a;
        decision = getfi(0, 0, 1, 0);
    else
        select_metric = b;
        decision = getfi(1, 0, 1, 0);
    end
end

function myfi = getfi(input, issigned, wlen, flen)

fm = fimath(...
    'RoundMode', 'floor',...
    'OverflowMode', 'wrap',...
    'ProductMode', 'FullPrecision', 'ProductWordLength', 32,...
    'SumMode', 'FullPrecision', 'SumWordLength', 32,...
    'CastBeforeSum', true);

myfi = fi(input, issigned, wlen, flen, 'fimath', fm);

end

== matlab function hdlcoderviterbi2/viterbi_eml_timed/TraceBack Unit/TBU5 ==
  settings: fimath=|
      | fimath(...
      | 'RoundMode', 'floor',...
      | 'OverflowMode', 'wrap',...
      | 'ProductMode', 'FullPrecision', 'ProductWordLength', 32,...
      | 'SumMode', 'FullPrecision', 'SumWordLength', 32,...
      | 'CastBeforeSum', true)
  data: dec input fixdt(0,1,0) size=[1 64]; index input fixdt(0,8,0) size=1; dec_out output; index_out output
function [dec_out, index_out] = TBU(dec, index)
%--------------------------------------------------------------------------
% TBU (Trace Back Unit)
% Trace back unit restore the optimal path information stored in the 
% path metric register. The trace back depth of this decoder is 32 steps,
% which means every decoded symbol is based on the minimum path metric in the
% following 32 steps. 
%
% The trace back unit is implemented by a 32 stage shift register.
% In this pipelined model, 32 stage shift register is breaked into 8 4-stage shift registers. 
%--------------------------------------------------------------------------

% initialize 4-stage trace back storage shift register
persistent tb_reg1 tb_reg2 tb_reg3 tb_reg4
if isempty(tb_reg1)
    tb_reg1 = getfi(zeros(1, 64), 0, 1, 0);
end
if isempty(tb_reg2)
    tb_reg2 = getfi(zeros(1, 64), 0, 1, 0);
end
if isempty(tb_reg3)
    tb_reg3 = getfi(zeros(1, 64), 0, 1, 0);
end
if isempty(tb_reg4)
    tb_reg4 = getfi(zeros(1, 64), 0, 1, 0);
end

% 4-stage trace back storage shift register
% stores path metric decision inforamtion from ACS unit
dec_out = tb_reg4;
tb_reg4 = tb_reg3;
tb_reg3 = tb_reg2;
tb_reg2 = tb_reg1;
tb_reg1 = dec;

% stage one
idx = int32(index) + int32(1);
tbread = tb_reg1(idx);
shift_idx = bitconcat(bitsliceget(index, 5, 1), tbread);
index = bitconcat(getfi(0, 0, 2, 0), shift_idx);

% stage two
idx = int32(index) + int32(1);
tbread = tb_reg2(idx);
shift_idx = bitconcat(bitsliceget(index, 5, 1), tbread);
index = bitconcat(getfi(0, 0, 2, 0), shift_idx);

% stage three
idx = int32(index) + int32(1);
tbread = tb_reg3(idx);
shift_idx = bitconcat(bitsliceget(index, 5, 1), tbread);
index = bitconcat(getfi(0, 0, 2, 0), shift_idx);

% stage four
idx = int32(index) + int32(1);
tbread = tb_reg4(idx);
shift_idx = bitconcat(bitsliceget(index, 5, 1), tbread);
index_out = bitconcat(getfi(0, 0, 2, 0), shift_idx);

end

function myfi = getfi(input, issigned, wlen, flen)

fm = fimath(...
    'RoundMode', 'floor',...
    'OverflowMode', 'wrap',...
    'ProductMode', 'FullPrecision', 'ProductWordLength', 32,...
    'SumMode', 'FullPrecision', 'SumWordLength', 32,...
    'CastBeforeSum', true);

myfi = fi(input, issigned, wlen, flen, 'fimath', fm);

end
